simulink model "ABS_Ctrl"  (R2022b)
settings: Solver=VariableStepAuto  StartTime=0.0  StopTime=10  RelTol=1e-3
model workspace (MAT data in the model file):
  ABS_BrkGainKf = Simulink.Parameter
  ABS_BrkGainKf.Value = 1500
  ABS_BrkGainKf.Description = 'Brake gain from pressure command to brake torque'
  ABS_BrkGainKf.DataType = 'auto'
  ABS_BrkGainKf.Min = 0
  ABS_BrkGainKf.Max = 5000
  ABS_BrkGainKf.DocUnits = 'N*m'
  ABS_BrkGainKf.Complexity = 'real'
  ABS_BrkGainKf.Dimensions = [1 1]
  ABS_HydrLagTb = Simulink.Parameter
  ABS_HydrLagTb.Value = 0.01
  ABS_HydrLagTb.Description = 'Time constant of the brake hydraulics'
  ABS_HydrLagTb.DataType = 'auto'
  ABS_HydrLagTb.Min = 0.001
  ABS_HydrLagTb.Max = 0.5
  ABS_HydrLagTb.DocUnits = 's'
  ABS_HydrLagTb.Complexity = 'real'
  ABS_HydrLagTb.Dimensions = [1 1]
  ABS_SlipRef = Simulink.Parameter
  ABS_SlipRef.Value = 0.2
  ABS_SlipRef.Description = 'Target wheel slip (near peak tire friction)'
  ABS_SlipRef.DataType = 'auto'
  ABS_SlipRef.Min = 0
  ABS_SlipRef.Max = 1
  ABS_SlipRef.DocUnits = '1'
  ABS_SlipRef.Complexity = 'real'
  ABS_SlipRef.Dimensions = [1 1]
  ABS_WhlRadius = Simulink.Parameter
  ABS_WhlRadius.Value = 0.3
  ABS_WhlRadius.Description = 'Dynamic wheel radius'
  ABS_WhlRadius.DataType = 'auto'
  ABS_WhlRadius.Min = 0.1
  ABS_WhlRadius.Max = 0.6
  ABS_WhlRadius.DocUnits = 'm'
  ABS_WhlRadius.Complexity = 'real'
  ABS_WhlRadius.Dimensions = [1 1]
Description:
  | Simplified ABS slip controller (bang-bang) for EHANDBOOK training.
settings Model: Creator=ZJO9FE  LastModifiedBy=ZJO9FE

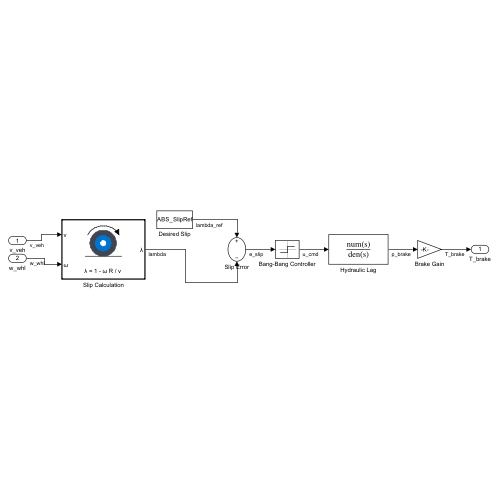
[thumbnail: Simulink's stored preview of the top-level diagram]
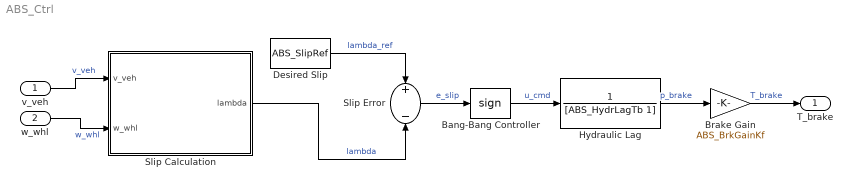
== system ABS_Ctrl ==
  v_veh : Inport  Unit=m/s
  w_whl : Inport  Port=2  Unit=rad/s
  Bang-Bang Controller : Signum  Description=+1: build up pressure, -1: release pressure
  Brake Gain : Gain  Description=Converts pressure command to brake torque  Gain=ABS_BrkGainKf
  Desired Slip : Constant  Description=Target slip reference  Value=ABS_SlipRef
  Hydraulic Lag : TransferFcn  Description=First-order lag of the brake hydraulics  Numerator=1  Denominator=[ABS_HydrLagTb 1]
  Slip Calculation : MATLAB Function  Description=Wheel slip lambda = 1 - w*R/v  TreatAsAtomicUnit=on  mask(Wheel Slip){}
      mask help: Computes the longitudinal wheel slip from vehicle speed and wheel speed.
  Slip Error : Sum  Description=e = lambda_ref - lambda  Inputs=+-
  T_brake : Outport  Unit=N*m
  wires:
  v_veh/1 -> Slip Calculation/1(v_veh)  "v_veh"
  w_whl/1 -> Slip Calculation/2(w_whl)  "w_whl"
  Desired Slip/1 -> Slip Error/1  "lambda_ref"
  Slip Calculation/1(lambda) -> Slip Error/2  "lambda"
  Slip Error/1 -> Bang-Bang Controller/1  "e_slip"
  Bang-Bang Controller/1 -> Hydraulic Lag/1  "u_cmd"
  Hydraulic Lag/1 -> Brake Gain/1  "p_brake"
  Brake Gain/1 -> T_brake/1  "T_brake"

== matlab function ABS_Ctrl/Slip Calculation ==
  data: v_veh input; lambda output; w_whl input; ABS_WhlRadius parameter
function lambda = slip_calc(v_veh, w_whl, ABS_WhlRadius)
%#codegen
% Guard against division by zero at standstill
v = max(v_veh, 0.1);
lambda = 1 - (w_whl * ABS_WhlRadius) / v;
